simulink model "tilt_closed_loop"  (R2024a)
settings: Solver=ode4  StartTime=0.0  StopTime=45  FixedStep=1e-3  RelTol=1e-3
settings Model: Creator=qixiaoyang  LastModifiedBy=qixiaoyang

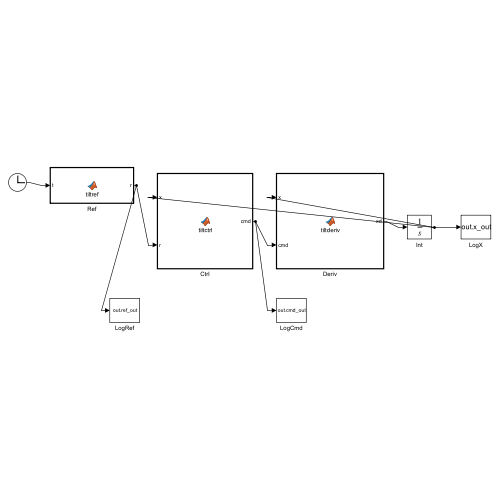
[thumbnail: Simulink's stored preview of the top-level diagram]
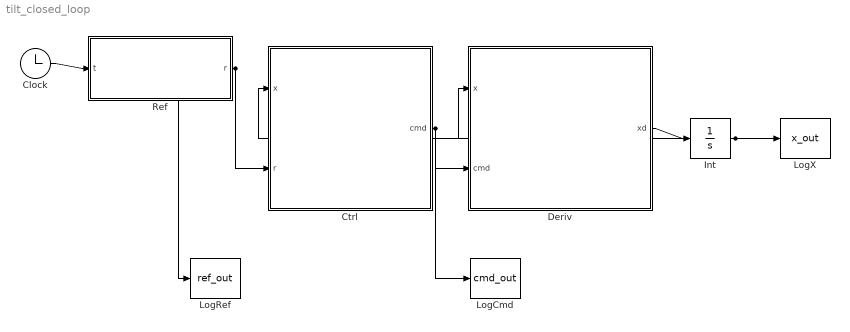
== system tilt_closed_loop ==
  Clock : Clock
  Ctrl : MATLAB Function  TreatAsAtomicUnit=on
  Deriv : MATLAB Function  TreatAsAtomicUnit=on
  Int : Integrator  InitialCondition=[0;0;-20;0;0;0;1;0;0;0;0;0;0;0;868.68601037163296;868.68601037163296;868.68601037163296;868.68601037163296;0;0;0]
  LogCmd : ToWorkspace  VariableName=cmd_out  SaveFormat=Timeseries  SampleTime=-1
  LogRef : ToWorkspace  VariableName=ref_out  SaveFormat=Timeseries  SampleTime=-1
  LogX : ToWorkspace  VariableName=x_out  SaveFormat=Timeseries  SampleTime=-1
  Ref : MATLAB Function  TreatAsAtomicUnit=on
  wires:
  Clock/1 -> Ref/1(t)
  Int/1 -> Ctrl/1(x), Deriv/1(x), LogX/1
  Ref/1(r) -> Ctrl/2(r), LogRef/1
  Ctrl/1(cmd) -> Deriv/2(cmd), LogCmd/1
  Deriv/1(xd) -> Int/1

== matlab function tilt_closed_loop/Ref ==
  data: t input; r output
function r = tiltref(t)
% 悬停-转捩-巡航任务参考，返回 [p(3); v(3); a(3); psi; h; V]
Vmax = 22;
Ta = 15;
t1 = 5;
t2 = 20;
h0 = 20;
pAcc = Vmax*Ta/2;
if t <= t1
    V = 0; aN = 0; pN = 0;
elseif t <= t2
    tau = t - t1;
    V  = Vmax/2*(1 - cos(pi*tau/Ta));
    aN = Vmax/2*(pi/Ta)*sin(pi*tau/Ta);
    pN = Vmax/2*(tau - (Ta/pi)*sin(pi*tau/Ta));
else
    V = Vmax; aN = 0; pN = pAcc + Vmax*(t - t2);
end
r = [pN; 0; -h0; V; 0; 0; aN; 0; 0; 0; h0; V];
end

== matlab function tilt_closed_loop/Deriv ==
  data: x input; xd output; cmd input
function xd = tiltderiv(x, cmd)
% 21 维导数：13 刚体 + 短舱 + 4 转速 + 3 舵面，含一阶滞后
Vb = x(4:6); q = x(7:10); w = x(11:13);
beta = x(14); om = x(15:18); act = x(19:21);
R = dcm(q);
u = Vb(1); vv = Vb(2); wb = Vb(3);
pp = w(1); qq = w(2); rr = w(3);
de = act(1); da = act(2); dr = act(3);
V = norm(Vb); Ve = max(V, 1.0);
alpha = asin(max(-0.34, min(0.34, wb/Ve)));
bsa = asin(max(-0.34, min(0.34, vv/Ve)));
qbar = 0.5*1.2250000000000001*V^2;
CL = 0.45000000000000001 + 5*alpha + 3.8999999999999999*qq*0.34000000000000002/(2*Ve) + 0.40000000000000002*de;
CD = 0.025000000000000001 + 0.044999999999999998*CL^2;
CY = -0.59999999999999998*bsa + 0.19*dr;
D = qbar*1.6000000000000001*CD; L = qbar*1.6000000000000001*CL; Y = qbar*1.6000000000000001*CY;
Xa = -D*cos(alpha) + L*sin(alpha);
Za = -D*sin(alpha) - L*cos(alpha);
Fa = [Xa; Y; Za];
Ma1 = qbar*1.6000000000000001*3.6000000000000001*(-0.089999999999999997*bsa + -0.5*pp*3.6000000000000001/(2*Ve) + 0.080000000000000002*rr*3.6000000000000001/(2*Ve) + 0.17999999999999999*da);
Ma2 = qbar*1.6000000000000001*0.34000000000000002*(0.050000000000000003 + -0.80000000000000004*alpha + -12*qq*0.34000000000000002/(2*Ve) + -1.2*de);
Ma3 = qbar*1.6000000000000001*3.6000000000000001*(0.059999999999999998*bsa + -0.029999999999999999*pp*3.6000000000000001/(2*Ve) + -0.12*rr*3.6000000000000001/(2*Ve) + 0.089999999999999997*dr);
Ma = [Ma1; Ma2; Ma3];
T = 2.5999999999999998e-05*om.^2;
U1 = sum(T);
U2 = -sum([[0.90000000000000002]; [0.90000000000000002]; [-0.90000000000000002]; [-0.90000000000000002]].*T);
U3 = sum([[0.40000000000000002]; [-0.40000000000000002]; [-0.40000000000000002]; [0.40000000000000002]].*T);
U4 = sum([[1]; [-1]; [1]; [-1]].*T);
sb = sin(beta); cb = cos(beta);
Fr = [sb; 0; -cb]*U1;
Mr = [cb*U2 - 0.019230769230769232*sb*U4; cb*U3; sb*U2 + 0.019230769230769232*cb*U4];
Fb = Fa + Fr;
Mb = Ma + Mr;
Vn = R*Vb;
Vbd = Fb/8 - cross(w, Vb) + R'*[0; 0; 9.8100000000000005];
qd = 0.5*qmul(q, [0; w]);
Imat = [0.90000000000000002 0 0; 0 1.2 0; 0 0 1.6000000000000001];
wd = Imat \ (Mb - cross(w, Imat*w));
betaDot = (cmd(8) - beta)/0.14999999999999999;
betaDot = min(max(betaDot, -0.52359877559829882), 0.52359877559829882);
omDot = (cmd(1:4) - om)/0.02;
actDot = (cmd(5:7) - act)/0.050000000000000003;
xd = [Vn; Vbd; qd; wd; betaDot; omDot; actDot];
end
function R = dcm(q)
n = norm(q);
if n < 1e-12, q = [1;0;0;0]; else, q = q/n; end
w = q(1); x = q(2); y = q(3); z = q(4);
R = [1-2*(y*y+z*z), 2*(x*y-w*z), 2*(x*z+w*y);
     2*(x*y+w*z), 1-2*(x*x+z*z), 2*(y*z-w*x);
     2*(x*z-w*y), 2*(y*z+w*x), 1-2*(x*x+y*y)];
end
function r = qmul(a, b)
aw = a(1); av = a(2:4);
bw = b(1); bv = b(2:4);
r = [aw*bw - av'*bv; aw*bv + bw*av + cross(av, bv)];
end

== matlab function tilt_closed_loop/Ctrl ==
  settings: updateMethod=DISCRETE  sampleTime=1e-3
  data: x input; cmd output; r input
function cmd = tiltctrl(x, r)
% 倾转四旋翼级联控制：位置环 -> 姿态混合 -> 权限分配
persistent ip ia iH
if isempty(ip)
    ip = zeros(3,1); ia = zeros(3,1); iH = 0;
end
dt = 0.001;
Vb = x(4:6);
q  = x(7:10);
w  = x(11:13);
beta = x(14);
act  = x(19:21);
R  = dcm(q);
att = euler(q);
psi = att(3);
Vn = R*Vb;
V  = norm(Vb);
alpha = atan2(Vb(3), Vb(1));
h = -x(3);
hdot = V*sin(att(2) - alpha);
qbar = 0.5*1.2250000000000001*V^2;
k = (min(V, r(12) + 2.0) - 3)/(14 - 3);
k = min(max(k, 0), 1);
ep = r(1:3) - x(1:3);
ev = r(4:6) - Vn;
ip = ip + ep*dt;
ip = min(max(ip, -[0;0;1.2]), [0;0;1.2]);
a = [1;1;1.6000000000000001].*ep + [1.8;1.8;2.2000000000000002].*ev + r(7:9) + [0;0;0.80000000000000004].*ip;
nh = norm(a(1:2));
if nh > 2.5
    a(1:2) = a(1:2)*(2.5/nh);
end
a(3) = min(max(a(3), -4), 4);
Vref = norm(r(4:6));
if V > Vref + 2 && V > 1
    ehat = Vn/V;
    along = a'*ehat;
    aCap = -(V - Vref - 2);
    if along > aCap
        a = a + ehat*(aCap - along);
    end
end
Tn = 8*(a - [0; 0; 9.8100000000000005]);
Tnb = R'*Tn;
Fa = aero(Vb, w, act);
Frot = Tnb - Fa;
if norm(Frot) < 1e-6
    Frot = [0; 0; -8*9.8100000000000005];
end
qbarS = max(qbar, 1.0);
CLreq = 8*9.8100000000000005/(qbarS*1.6000000000000001);
alphaT = (CLreq - 0.45000000000000001)/5;
alphaT = min(max(alphaT, -0.20000000000000001), 0.29999999999999999);
alphaT = k*alphaT;
zq = -Tn/max(norm(Tn), 1e-9);
xc = [cos(psi); sin(psi); 0];
yb = cross(zq, xc);
ny = norm(yb);
if ny < 1e-6
    xc = [1; 0; 0];
    yb = cross(zq, xc);
    ny = norm(yb);
end
yb = yb/ny;
xb = cross(yb, zq);
Rdq = [xb yb zq];
phiQ = atan2(Rdq(3,2), Rdq(3,3));
thetaQ = -asin(min(max(Rdq(3,1), -1), 1));
eH = r(11) - h;
iH = iH + eH*dt;
iH = min(max(iH, -40), 40);
thetaF = alphaT + 0.029999999999999999*eH + 0.0060000000000000001*iH - 0.040000000000000001*hdot + 0.029999999999999999*(V - r(12));
thetaF = min(max(thetaF, -0.29999999999999999), 0.29999999999999999);
ePsi = mod(r(10) - psi + pi, 2*pi) - pi;
phiF = 0.80000000000000004*ePsi;
phiF = min(max(phiF, -0.45000000000000001), 0.45000000000000001);
phiD   = (1 - k)*phiQ + k*phiF;
thetaD = (1 - k)*thetaQ + k*thetaF;
psiD   = r(10);
eAtt = mod([phiD; thetaD; psiD] - att + pi, 2*pi) - pi;
ia = ia + eAtt*dt;
ia = min(max(ia, -[0;0;0.34999999999999998]), [0;0;0.34999999999999998]);
Mraw = [6;6;3].*eAtt + [0;0;0.59999999999999998].*ia - [4;4;2].*w;
wRot0 = max(0, 1 - k);
gb = max(1, max(qbar, 1.0)/20);
M = wRot0*Mraw + (1 - wRot0)*gb*Mraw;
MfLim = [qbar*1.6000000000000001*3.6000000000000001*0.17999999999999999*0.3490658503988659; qbar*1.6000000000000001*0.34000000000000002*1.2*0.43633231299858238; qbar*1.6000000000000001*3.6000000000000001*0.089999999999999997*0.43633231299858238];
Mlim = wRot0*[2.5;2.5;1] + (1 - wRot0)*MfLim;
M = min(max(M, -Mlim), Mlim);
sb = sin(beta); cb = cos(beta);
d = [sb; 0; -cb];
U1max = 4*2.5999999999999998e-05*1100^2;
U1v = norm(Frot);
U1f = max(0, d'*Frot);
U1 = max(0, min(U1max, (1 - k)*U1v + k*U1f));
wRot = max(0, 1 - k);
Mxr = wRot*M(1); Myr = wRot*M(2); Mzr = wRot*M(3);
U2 = cb*Mxr + sb*Mzr;
U3 = Myr/max(cb, 0.20);
U4 = (-sb*Mxr + cb*Mzr)/0.019230769230769232;
T1 = 0.25*U1 - 0.25*U2/0.90000000000000002 + 0.25*U3/0.40000000000000002 + 0.25*U4;
T2 = 0.25*U1 - 0.25*U2/0.90000000000000002 - 0.25*U3/0.40000000000000002 - 0.25*U4;
T3 = 0.25*U1 + 0.25*U2/0.90000000000000002 - 0.25*U3/0.40000000000000002 + 0.25*U4;
T4 = 0.25*U1 + 0.25*U2/0.90000000000000002 + 0.25*U3/0.40000000000000002 - 0.25*U4;
T = [T1; T2; T3; T4];
om = sqrt(max(T, 0)/2.5999999999999998e-05);
om = min(om, 1100);
qs = max(qbar, 1.0);
da = (1 - wRot)*M(1)/(qs*1.6000000000000001*3.6000000000000001*0.17999999999999999);
de = (1 - wRot)*M(2)/(qs*1.6000000000000001*0.34000000000000002*-1.2);
dr = (1 - wRot)*M(3)/(qs*1.6000000000000001*3.6000000000000001*0.089999999999999997);
actCmd = [min(max(de, -0.43633231299858238), 0.43633231299858238); min(max(da, -0.3490658503988659), 0.3490658503988659); min(max(dr, -0.43633231299858238), 0.43633231299858238)];
betaCmd = 0 + (1.5707963267948966 - 0)*k;
cmd = [om(:); actCmd(:); betaCmd];
end
function Fa = aero(Vb, w, act)
% 机体系气动力，act = [de; da; dr]，油门项为 0
u = Vb(1); v = Vb(2); wb = Vb(3);
pp = w(1); qq = w(2); rr = w(3);
de = act(1); da = act(2); dr = act(3);
V = norm(Vb); Ve = max(V, 1.0);
alpha = asin(max(-0.34, min(0.34, wb/Ve)));
bsa = asin(max(-0.34, min(0.34, v/Ve)));
qbar = 0.5*1.2250000000000001*V^2;
CL = 0.45000000000000001 + 5*alpha + 3.8999999999999999*qq*0.34000000000000002/(2*Ve) + 0.40000000000000002*de;
CD = 0.025000000000000001 + 0.044999999999999998*CL^2;
CY = -0.59999999999999998*bsa + 0.19*dr;
D = qbar*1.6000000000000001*CD; L = qbar*1.6000000000000001*CL; Y = qbar*1.6000000000000001*CY;
Xa = -D*cos(alpha) + L*sin(alpha);
Za = -D*sin(alpha) - L*cos(alpha);
Fa = [Xa; Y; Za];
end
function R = dcm(q)
n = norm(q);
if n < 1e-12, q = [1;0;0;0]; else, q = q/n; end
w = q(1); x = q(2); y = q(3); z = q(4);
R = [1-2*(y*y+z*z), 2*(x*y-w*z), 2*(x*z+w*y);
     2*(x*y+w*z), 1-2*(x*x+z*z), 2*(y*z-w*x);
     2*(x*z-w*y), 2*(y*z+w*x), 1-2*(x*x+y*y)];
end
function e = euler(q)
n = norm(q);
if n < 1e-12, e = [0;0;0]; return; end
q = q/n;
w = q(1); x = q(2); y = q(3); z = q(4);
s2 = 2*(w*y - z*x);
s2 = max(-1, min(1, s2));
e = [atan2(2*(w*x + y*z), 1 - 2*(x*x + y*y));
     asin(s2);
     atan2(2*(w*z + x*y), 1 - 2*(y*y + z*z))];
end
